simulink model "hybridModel3_2"  (R2025a)
settings: Solver=VariableStepAuto  StartTime=0.0  StopTime=180.0  RelTol=1e-3
InitFcn:
  | [p,x0] = hybridParams();
undefined symbols (not defined in the file): p, x0
settings Model: Creator=steen  LastModifiedBy=steen

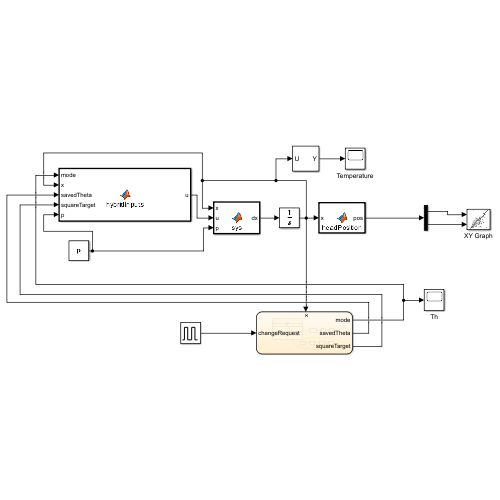
[thumbnail: Simulink's stored preview of the top-level diagram]
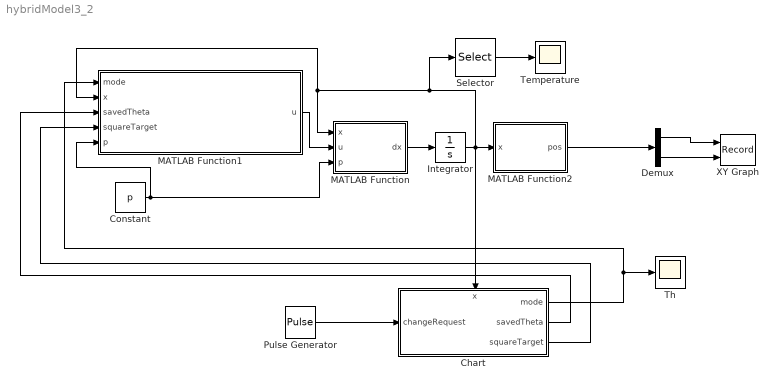
== system hybridModel3_2 ==
  Chart : Stateflow chart  TreatAsAtomicUnit=on
      settings: PortSchema="{\"entries\":[{\"content\":{\"sides\":[{\"content\":{\"connectorIds\":[\"In1\"]},\"type\":\"ConnectorPlacement.EquallySpacedRectSide\",\"uuid\":\"e4d83405-6ab7-42ad-8c2d-f12deafa8773\"},{\"content\":{\"connectorIds\":[\"Out1\",\"Out2\",\"Out3\"],\"side\":\"RIGHT\"},\"type\":\"ConnectorPlacement.EquallySpacedRectSide\",\"uuid\":\"897ea72c-623b-4d81-bbe9-567f5b8fd76a\"},{\"content\":{\"connectorIds\":[\"In2\"],\"side\":\"TOP\"},\"type\":\"ConnectorPlacement.EquallySpacedRectSide\",\"uuid\":\"51c51758-6a3d-420c-b6a4-8d2e35e362a2\"}]},\"type\":\"ConnectorPlacement.EquallySpacedConnector\",\"uuid\":\"b6a753e5-4678-4037-b7da-54d4882a2331\"}],\"packageUris\":[\"http://schema.mathworks.com/mf0/Connector/R2020b\"],\"version\":\"1.0\"}"
  Constant : Constant  Value=p
  Demux : Demux  Outputs=2
  Integrator : Integrator  InitialCondition=x0
  MATLAB Function : MATLAB Function  TreatAsAtomicUnit=on
  MATLAB Function1 : MATLAB Function  TreatAsAtomicUnit=on
  MATLAB Function2 : MATLAB Function  TreatAsAtomicUnit=on
  Pulse Generator : DiscretePulseGenerator  PulseType=Time based  Amplitude=0  Period=200  PulseWidth=0.5  PhaseDelay=2
  Selector : Selector  InputPortWidth=9  IndexOptions=Index vector (dialog)  Indices=9  OutputSizes=1
  Temperature : Scope
      settings: ActiveDisplayYMinimum=-51.618945788613033  ActiveDisplayYMaximum=368.28539455177713  DataLoggingVariableName=ScopeData2
  Th : Scope
      settings: ActiveDisplayYMinimum=-0.87499999999999978  ActiveDisplayYMaximum=7.875
  XY Graph : Record  NumPorts=2.0  FileSettingsInternal="{\"entries\":[{\"content\":{\"excelSettings\":{\"content\":{},\"type\":\"Streamout.ExcelSettings\"},\"parquetSettings\":{\"content\":{},\"type\":\"Streamout.ParquetSettings\"}},\"type\":\"Streamout.FileSettingStorage\",\"uuid\":\"\"}],\"packageUris\":[\"http:\\/\\/schema.mathworks.com\\/mf0\\/streamout_blocks\\/R2020a\"],\"version\":\"1.0\"}"  FrameSettings=[0, 0]  Layout=[1 1]  SignalsInternal="{\"entries\":[{\"content\":{\"signals\":[{\"content\":{\"blockPath\":[],\"dimensions\":[1,1],\"domain\":\"\",\"lineColor\":\"#a2142f\",\"plots\":[ 1 ],\"port\":1,\"sid\":[\"\"],\"signalID\":1,\"signalName\":\"Demux:1\"},\"type\":\"RecordBlkView.Signal\",\"uuid\":\"\"},{\"content\":{\"blockPath\":[],\"dimensions\":[1,1],\"domain\":\"\",\"lineColor\":\"#139fff\",\"plots\":[ 1 ],\"port\":2,\"sid\":[\"\"],\"signalID\":2,\"signalName\":\"Demux:2\"},\"type\":\"RecordBlkView.Signal\",\"uuid\":\"\"}]},\"type\":\"RecordBlkView.InputSignals\",\"uuid\":\"\"}],\"packageUris\":[\"http:\\/\\/schema.mathworks.com\\/mf0\\/streamout_blocks\\/R2020a\"],\"version\":\"1.0\"}"  VisualizationBindings="{\"xyplotplugin\":{\"info\":[{\"series\":[{\"bindingParametersList\":[{\"parameter\":\"X-Axis\",\"signalID\":1,\"signalName\":\"Demux:1\"},{\"parameter\":\"Y-Axis\",\"signalID\":2,\"signalName\":\"Demux:2\"}],\"seriesID\":0}],\"subplotID\":1}]}}"  CompatibilityTag=XY
  wires:
  Constant/1 -> MATLAB Function/3(p), MATLAB Function1/5(p)
  MATLAB Function/1(dx) -> Integrator/1
  Integrator/1 -> MATLAB Function2/1(x), Selector/1, MATLAB Function/1(x), MATLAB Function1/2(x), Chart/2(x)
  Pulse Generator/1 -> Chart/1(changeRequest)
  Chart/1(mode) -> MATLAB Function1/1(mode), Th/1
  MATLAB Function1/1(u) -> MATLAB Function/2(u)
  Chart/2(savedTheta) -> MATLAB Function1/3(savedTheta)
  MATLAB Function2/1(pos) -> Demux/1
  Selector/1 -> Temperature/1
  Chart/3(squareTarget) -> MATLAB Function1/4(squareTarget)
  Demux/1 -> XY Graph/1
  Demux/2 -> XY Graph/2

== matlab function hybridModel3_2/MATLAB Function1 ==
  data: mode input; u output; x input; savedTheta input; squareTarget input; p input
function u = hybridInputs(mode,x,savedTheta,squareTarget,p)

u = zeros(3,1);

if mode == 0
    target = squareTarget;
elseif mode == 2
    target = [0;0];
elseif mode == 7
    target = savedTheta;
else
    target = x(1:2);
end

if mode == 0 || mode == 2 || mode == 7
    Kp = 0.15;
    Kd = 0.025;

    error = target - x(1:2);
    u(1:2) = Kp*error - Kd*x(3:4);
    u(1:2) = max(-24,min(24,u(1:2)));
end

Rn = p(9);
Rt = p(11);
Te = p(12);

Vhold = sqrt(Rn*(200-Te)/Rt);

if mode == 4 || mode == 5
    u(3) = 0;
elseif mode == 6
    u(3) = 24;
else
    u(3) = Vhold;
end

end

== matlab function hybridModel3_2/MATLAB Function ==
  data: x input; u input; dx output; p input

function dx = sys(x,u,p)

J = p(1);
B11 = p(2);
B12 = p(3);
Km = p(4);
Lm = p(5);
Rm = p(6);

Ln = p(7);
Cn = p(8);
Rn = p(9);
Ct = p(10);
Rt = p(11);
Te = p(12);

dx = zeros(9,1);

dx(1) = x(3);
dx(2) = x(4);

dx(3) = (Km*x(5)-B11*x(3)-B12*x(4))/J;
dx(4) = (Km*x(6)-B12*x(3)-B11*x(4))/J;

dx(5) = (u(1)-Rm*x(5)-Km*x(3))/Lm;
dx(6) = (u(2)-Rm*x(6)-Km*x(4))/Lm;

dx(7) = (u(3)-x(8))/Ln;
dx(8) = (x(7)-x(8)/Rn)/Cn;
dx(9) = (x(8)^2/Rn-(x(9)-Te)/Rt)/Ct;

end

== stateflow chart hybridModel3_2/Chart ==
  state Printing
    entry:
    mode = 0;
    state entry_2
      squareTarget = [0.22/0.006; 0.10/0.006];
    state entry_3
      squareTarget = [0.28/0.006; 0.04/0.006];
    state entry_
      squareTarget = [0.16/0.006; 0.04/0.006];
    state entry_4
      squareTarget = [0.22/0.006; -0.02/0.006];
    (default) -> entry_2
    entry_2 -> entry_3 : [abs(x(1)-squareTarget(1))<0.05 && ...
        |  abs(x(2)-squareTarget(2))<0.05 && ...
        |  abs(x(3))<0.1 && abs(x(4))<0.1]
    entry_3 -> entry_4 : [abs(x(1)-squareTarget(1))<0.05 && ...
        |  abs(x(2)-squareTarget(2))<0.05 && ...
        |  abs(x(3))<0.1 && abs(x(4))<0.1]
    entry_4 -> entry_ : [abs(x(1)-squareTarget(1))<0.05 && ...
        |  abs(x(2)-squareTarget(2))<0.05 && ...
        |  abs(x(3))<0.1 && abs(x(4))<0.1]
  state StopSave
    entry:
    mode = 1;
    savedTheta = x(1:2);
  state Origin
    entry:
    mode = 2;
  state Wipe
    entry:
    mode = 3;
  state HeatOff
    entry:
    mode = 4;
  state Load
    entry:
    mode = 5;
  state HeatOn
    entry:
    mode = 6;
  state Return
    entry:
    mode = 7;
  (default) -> Printing
  StopSave -> Origin : [abs(x(3)) < 0.01 && abs(x(4)) < 0.01]
  Origin -> Wipe : [abs(x(1)) < 0.05 && abs(x(2)) < 0.05 && ...
      |  abs(x(3)) < 0.1 && abs(x(4)) < 0.1]
  Printing -> StopSave : [changeRequest]
  Wipe -> HeatOff : after(1,sec)
  Return -> Printing : [abs(x(1)-savedTheta(1)) < 0.05 && ...
      |  abs(x(2)-savedTheta(2)) < 0.05 && ...
      |  abs(x(3)) < 0.1 && abs(x(4)) < 0.1]
  HeatOn -> Return : [x(9) >= 200]
  HeatOff -> Load : [x(9) <= 80]
  Load -> HeatOn : after(1,sec)
  data: mode output; changeRequest input; x input; savedTheta output; squareTarget output

== matlab function hybridModel3_2/MATLAB Function2 ==
  data: x input; pos output
function pos = headPosition(x)

rm = 0.006;

pos = rm/2 * [x(1)+x(2); x(1)-x(2)];

end
